simulink model "modele_charriot"  (R2026a)
settings: Solver=FixedStepAuto  StopTime=20  FixedStep=1/100
values from neighbouring files (symbols this model uses):
  g = 9.81    [parametres_TP_chariot.m]
  masse = 15    [parametres_TP_chariot.m]
  mu = 0.18    [parametres_TP_chariot.m]
settings Model: Creator=lulu1  LastModifiedBy=lulu1

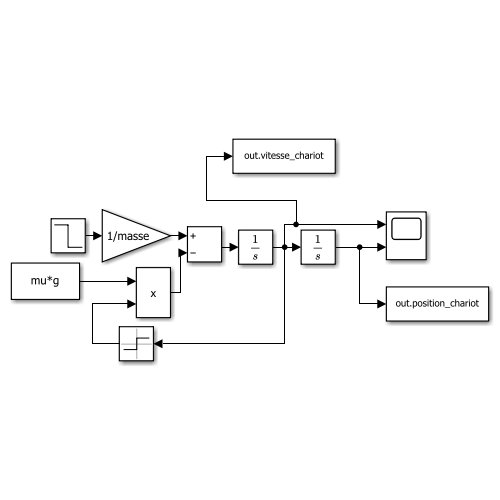
[thumbnail: Simulink's stored preview of the top-level diagram]
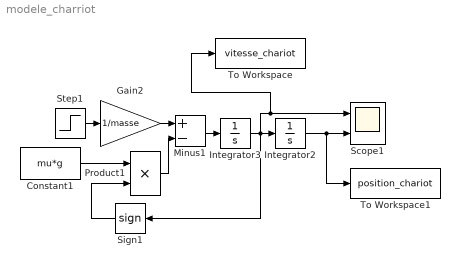
== system modele_charriot ==
  Constant1 : Constant  Value=mu*g
  Gain2 : Gain  Gain=1/masse
  Integrator2 : Integrator
  Integrator3 : Integrator
  Minus1 : Sum  Inputs=+-
  Product1 : Product
  Scope1 : Scope  NumInputPorts=2
      settings: ActiveDisplayYMinimum=-0.2906847467076657  ActiveDisplayYMaximum=2.3720295390066144
  Sign1 : Signum
  Step1 : Step  Time=10  InitialValue=F_pousse  FinalValue=0  SampleTime=0
  To Workspace : ToWorkspace  VariableName=vitesse_chariot  SaveFormat=Timeseries  SampleTime=-1
  To Workspace1 : ToWorkspace  VariableName=position_chariot  SaveFormat=Timeseries  SampleTime=-1
  wires:
  Integrator3/1 -> To Workspace/1, Scope1/1, Sign1/1, Integrator2/1
  Integrator2/1 -> To Workspace1/1, Scope1/2
  Gain2/1 -> Minus1/1
  Minus1/1 -> Integrator3/1
  Product1/1 -> Minus1/2
  Constant1/1 -> Product1/1
  Sign1/1 -> Product1/2
  Step1/1 -> Gain2/1
